simulink model "DebouncePlantModel_Harness1"  (R2024b)
settings: Solver=VariableStepAuto  StartTime=0.0  StopTime=5  RelTol=1e-3
settings Model: Creator=User  LastModifiedBy=User

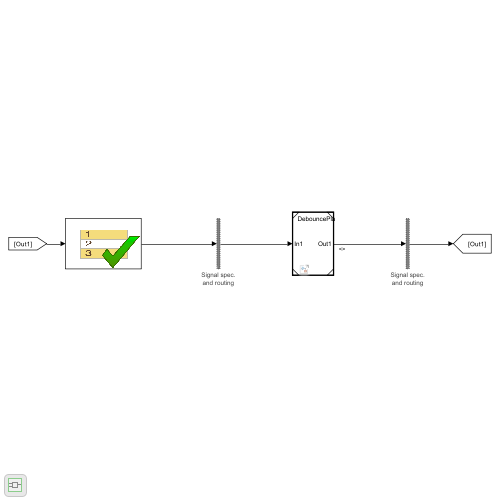
[thumbnail: Simulink's stored preview of the top-level diagram]
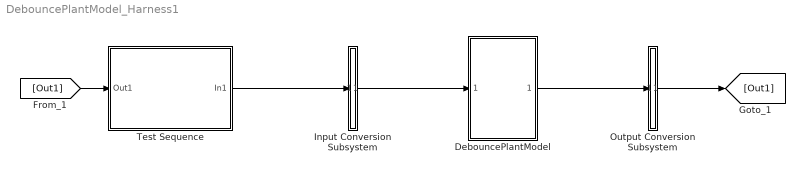
== system DebouncePlantModel_Harness1 ==
  DebouncePlantModel : ModelReference  ModelNameDialog=DebouncePlantModel  SimulationMode=Normal  ModelReferenceVersion=1.2
  Input Conversion Subsystem : Subsystem  Tag=__SLT_ICS__  Description=|
      | Signal spec.
      | and routing
      settings: AttributesFormatString=%<Description>
  Output Conversion Subsystem : Subsystem  Tag=__SLT_OCS__  Description=|
      | Signal spec.
      | and routing
      settings: AttributesFormatString=%<Description>
  Test Sequence : Test Sequence  TreatAsAtomicUnit=on
  wires:
  Test Sequence/1(In1) -> Input Conversion Subsystem/1(Inport_1)
  [Out1] -> Test Sequence/1(Out1)
  Output Conversion Subsystem/1(Outport_1) -> [Out1]
  Input Conversion Subsystem/1(Outport_1) -> DebouncePlantModel/1
  DebouncePlantModel/1 -> Output Conversion Subsystem/1(Inport_1)

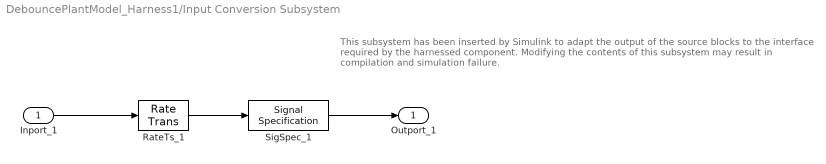
== system DebouncePlantModel_Harness1/Input Conversion Subsystem ==
  note: This subsystem has been inserted by Simulink to adapt the output of the source blocks to the interface required by the harnessed component.
      |  Modifying the contents of this subsystem may result in compilation and simulation failure.
  Inport_1 : Inport
  RateTs_1 : RateTransition  OutPortSampleTime=0.001
  SigSpec_1 : SignalSpecification  OutDataTypeStr=double  Dimensions=[1]  SampleTime=0.001
  Outport_1 : Outport
  wires:
  SigSpec_1/1 -> Outport_1/1
  RateTs_1/1 -> SigSpec_1/1
  Inport_1/1 -> RateTs_1/1

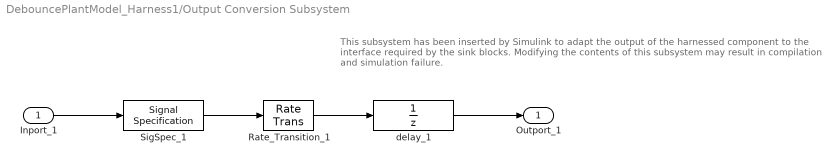
== system DebouncePlantModel_Harness1/Output Conversion Subsystem ==
  note: This subsystem has been inserted by Simulink to adapt the output of the harnessed component to the interface required by the sink blocks.
      |  Modifying the contents of this subsystem may result in compilation and simulation failure.
  Inport_1 : Inport
  Rate_Transition_1 : RateTransition  OutPortSampleTimeOpt=Inherit
  SigSpec_1 : SignalSpecification  OutDataTypeStr=boolean  Dimensions=[1]  SampleTime=0.001
  delay_1 : UnitDelay  SampleTime=-1
  Outport_1 : Outport
  wires:
  Inport_1/1 -> SigSpec_1/1
  SigSpec_1/1 -> Rate_Transition_1/1
  Rate_Transition_1/1 -> delay_1/1
  delay_1/1 -> Outport_1/1

== stateflow chart DebouncePlantModel_Harness1/Test Sequence ==
  state Scenario_1
    state Run
      %% Initialize data outputs.
      In1 = 1;
    (default) -> Scenario_1.Run
  state Scenario_2
    state Run
      %% Initialize data outputs.
      In1 = 0;
    state step_1
      In1 = 1;
    state step_2
      In1 = 0;
    state step_3
      In1 = 1;
    state step_4
      In1 = 0;
    state step_5
      In1 = 1;
    state step_6
      In1 = 1;
    state step_7
      In1 = 0;
    state step_8
      In1 = 1;
    state step_9
      In1 = 0;
    (default) -> Scenario_2.Run
    Scenario_2.Run -> step_1 : [
        | after(1,msec)
        | ]
    step_1 -> step_2 : [
        | after(1,msec)
        | ]
    step_2 -> step_3 : [
        | after(1,msec)
        | ]
    step_3 -> step_4 : [
        | after(1,msec)
        | ]
    step_4 -> step_5 : [
        | after(1,msec)
        | ]
    step_5 -> step_6 : [
        | after(51,msec)
        | ]
    step_6 -> step_7 : [
        | after(5,msec)
        | ]
    step_7 -> step_6 : [
        | after(10,msec)
        | ]
    step_8 -> step_7 : [
        | after(51,msec)
        | ]
  (default) -> Scenario_1 [order 1] : [Active_Scenario_Index == 1]
  (default) -> Scenario_2 [order 2] : {assert(Active_Scenario_Index == 2,'The value of Scenario Parameter ''Active_Scenario_Index'' is not valid. Use the index of the scenario to specify it.')}
  data: Out1 input boolean size=[1]; In1 output double size=[1]; Active_Scenario_Index parameter =2
